simulink library "NodeLib"  (R2025b)
settings: Solver=VariableStepAuto  StartTime=0.0  StopTime=10.0  RelTol=1e-3
settings Model: Creator=jjha  LastModifiedBy=jjha

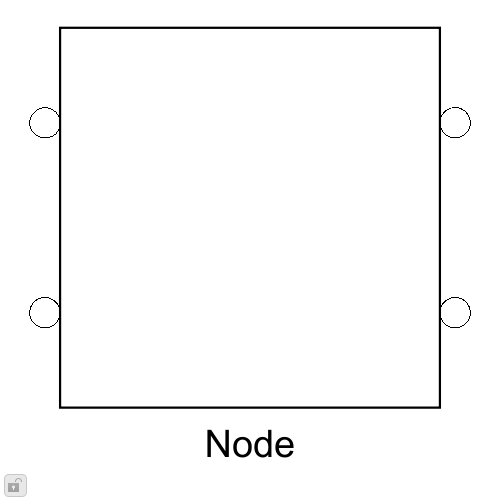
[thumbnail: Simulink's stored preview of the top-level diagram]
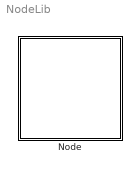
== system NodeLib ==
  Node : Subsystem

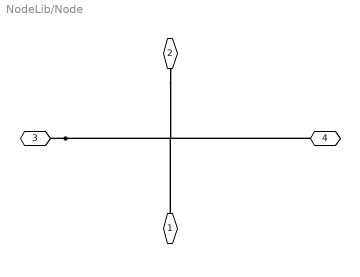
== system NodeLib/Node ==
  "   " : PMIOPort  Side=Left
  " " : PMIOPort  Port=2  Side=Left
  "  " : PMIOPort  Port=3  Side=Right
  "    " : PMIOPort  Port=4  Side=Right
  connections:
  "  "/RConn1 -- "   "/RConn1 -- "    "/RConn1 -- " "/RConn1
